simulink model "System_D_frequency_sweep"  (R2026a)
settings: Solver=ode23t  StopTime=1.45  MaxStep=1/(2*fs)  RelTol=1e-5
PostLoadFcn:
  | addpath(fileparts(get_param(bdroot,'FileName')));
InitFcn:
  | evalin('base','clear system_d_sweep_log system_d_frequency_response'); close(findall(groot,'Type','figure','Tag','SystemDFrequencyResponse'));
StopFcn:
  | plot_frequency_sweep(bdroot);
model workspace (MAT data in the model file):
  Cmid = 6.8e-06
  Ctw = 5.6e-06
  Lmid = 0.00082
  Ltw = 0.00022
  Rp = 3.3
  Rs = 4.7
  a_hp = [1 -1.96992019814 0.970365941122]
  a_lp = [1 -1.96992019814 0.970365941122]
  b_hp = [0.985071534816 -1.97014306963 0.985071534816]
  b_lp = [0.000111435745339 0.000222871490678 0.000111435745339]
  delay_samples = 16384
  f = [50 51 52 53 54 55 56 57 58 59 60 61 ... (412 elements, 412x1)]
  fir_mid = [2.88615785051e-06 2.87905807458e-06 2.86601289236e-06 2.86209989692e-06 2.87914488669e-06 2.90760278468e-06 2.91495292008e-06 2.86191467289e-06 2.72461541069e-06 2.51079055348e-06 2.26185413326e-06 2.03723101733e-06 ... (32768 elements, 1x32768)]
  fir_tw = [-2.60624232609e-06 -2.27215528381e-06 -2.25731305883e-06 -2.5961984087e-06 -2.98688820194e-06 -3.09958236215e-06 -2.8639414963e-06 -2.40425500843e-06 -1.83630123021e-06 -1.24253482671e-06 -7.49249289368e-07 -4.94473143896e-07 ... (32768 elements, 1x32768)]
  fir_woof = [2.71744577313e-06 2.91995199079e-06 3.2994659548e-06 3.73731262893e-06 4.11733049488e-06 4.36319861388e-06 4.44606576447e-06 4.38093146601e-06 4.22485207588e-06 4.06866670403e-06 4.00752757287e-06 4.09493136226e-06 ... (32768 elements, 1x32768)]
  fs = 96000
  g_woof = 0.595662143529
  pol_mid = 1
  pol_tw = 1
  pol_woof = 1
  ref_mid_im = [-2.02471473106e-05 -2.97451137892e-05 -8.18998441469e-06 -9.44112206059e-06 -9.98474521822e-06 -1.80323069699e-05 -2.36335585807e-05 -2.07669965717e-05 -2.44493768902e-05 1.53522925063e-05 1.26835054665e-05 -2.72017381443e-05 ... (412 elements, 412x1)]
  ref_mid_re = [5.11138743346e-05 5.27646175102e-05 6.43853406534e-05 7.19878043236e-05 9.07552490467e-05 9.02364974629e-05 0.000108111340774 0.000127641838401 0.000164076149146 0.00016525070791 0.000233272470596 0.000266015581949 ... (412 elements, 412x1)]
  ref_sum_im = [-0.237822623935 -0.249208923528 -0.252704050496 -0.277443609145 -0.287425433384 -0.281925307353 -0.273684166346 -0.301968651196 -0.32702532988 -0.356393021871 -0.384013551582 -0.427201303434 ... (412 elements, 412x1)]
  ref_sum_re = [0.0079461204201 -0.00807298700672 0.0366054479648 0.0304994442536 0.00185490294456 0.00396661293164 0.0289494720887 0.0412739478932 0.0471470600314 0.0668622907578 0.0743628077169 0.0739295887598 ... (412 elements, 412x1)]
  ref_tw_im = [2.66562025616e-10 1.06047214067e-10 3.29547259586e-10 9.1080418365e-11 1.01471933591e-10 -1.2721995912e-10 -3.07463357353e-10 -9.90286820009e-10 -4.40391607082e-10 -7.61622541983e-10 -4.0356932662e-10 2.86227803489e-10 ... (412 elements, 412x1)]
  ref_tw_re = [-2.81565378421e-10 4.5611348125e-11 -1.70188531961e-10 -5.4214307034e-11 1.59527809471e-12 1.81051243455e-11 4.85092069489e-10 1.65769684723e-11 -4.00879085044e-10 1.05530110859e-10 -9.04825296789e-10 -1.29396251722e-09 ... (412 elements, 412x1)]
  ref_woof_im = [-0.237802377054 -0.24917917852 -0.252695860841 -0.277434168114 -0.28741544874 -0.281907274919 -0.27366053248 -0.301947883209 -0.327000880063 -0.356408373402 -0.384026234684 -0.427174101982 ... (412 elements, 412x1)]
  ref_woof_re = [0.00789500682733 -0.00812575166984 0.0365410627943 0.0304274565035 0.00176414769392 0.00387637641607 0.0288413602628 0.0411463060382 0.0469829842831 0.0666970399443 0.0741295361511 0.0736635744718 ... (412 elements, 412x1)]
  sweep_input = [0 1.04166666667e-05 2.08333333333e-05 3.125e-05 4.16666666667e-05 5.20833333333e-05 6.25e-05 7.29166666667e-05 8.33333333333e-05 9.375e-05 0.000104166666667 0.000114583333333 ... (278402 elements, 139201x2)]
  tf_mid = [0.0998356483895 0.102076870231 0.0946421894936 0.0979510358274 0.112990905181 0.109044667147 0.122419200152 0.130377482303 0.15467322795 0.125179778541 0.168395608846 0.197284206678 ... (412 elements, 412x1)]
  tf_mid_im = [0.00966008754272 -0.00313844645705 0.0361663561834 0.0379690093634 0.0477044018154 0.03621348334 0.0393998382701 0.0511658321292 0.064682478583 0.0942375054511 0.119101574545 0.0996824269753 ... (412 elements, 412x1)]
  tf_mid_re = [0.0998356483895 0.102076870231 0.0946421894936 0.0979510358274 0.112990905181 0.109044667147 0.122419200152 0.130377482303 0.15467322795 0.125179778541 0.168395608846 0.197284206678 ... (412 elements, 412x1)]
  tf_tw = [0.0198457022563 8.34206280492e-05 0.012563148971 0.00336856881883 0.00145980497416 -0.00222599627599 -0.0157604599169 -0.0116189930625 0.00333344091506 -0.00916110563484 0.0108979357018 0.0209366637571 ... (412 elements, 412x1)]
  tf_tw_im = [-0.00715469241983 -0.00557696831399 -0.00982739097113 -0.00227734746733 -0.00315933910186 0.00326018180298 0.00155018479379 0.0216379610708 0.0128808016901 0.0125093739866 0.0144059793721 0.00636489608235 ... (412 elements, 412x1)]
  tf_tw_re = [0.0198457022563 8.34206280492e-05 0.012563148971 0.00336856881883 0.00145980497416 -0.00222599627599 -0.0157604599169 -0.0116189930625 0.00333344091506 -0.00916110563484 0.0108979357018 0.0209366637571 ... (412 elements, 412x1)]
  tf_woof = [0.181608417788 0.168786108916 0.242166050712 0.254795120302 0.223128594979 0.225804856879 0.259960687795 0.304360000511 0.337174588175 0.394426682217 0.432789825657 0.473682687703 ... (412 elements, 412x1)]
  tf_woof_im = [-0.356022917871 -0.383280529798 -0.354017107262 -0.393610885978 -0.428249167557 -0.416417838149 -0.382374342555 -0.411814390306 -0.441052500026 -0.464522244478 -0.494799805707 -0.553647303077 ... (412 elements, 412x1)]
  tf_woof_re = [0.181608417788 0.168786108916 0.242166050712 0.254795120302 0.223128594979 0.225804856879 0.259960687795 0.304360000511 0.337174588175 0.394426682217 0.432789825657 0.473682687703 ... (412 elements, 412x1)]
  zi_mid_im = [3.15145569017 3.226811686 3.32611598161 3.44333048105 3.54533776416 3.64854828115 3.76283446092 3.89289495957 4.01551140677 4.150592994 4.29260801654 4.46368784868 ... (412 elements, 412x1)]
  zi_mid_re = [5.31943483026 5.378404173 5.39638717148 5.47983267484 5.52299089563 5.59239183084 5.67547146448 5.74779130072 5.80510938691 5.884400566 5.98099909956 6.07160964327 ... (412 elements, 412x1)]
  zi_tw_im = [0.3929867032 0.3929867032 0.3929867032 0.3929867032 0.3929867032 0.3929867032 0.3929867032 0.3929867032 0.3929867032 0.3929867032 0.3929867032 0.3929867032 ... (412 elements, 412x1)]
  zi_tw_re = [3.639639303 3.639639303 3.639639303 3.639639303 3.639639303 3.639639303 3.639639303 3.639639303 3.639639303 3.639639303 3.639639303 3.639639303 ... (412 elements, 412x1)]
libraries: fl_lib x25, nesl_utility x5
(part 2 of 2)

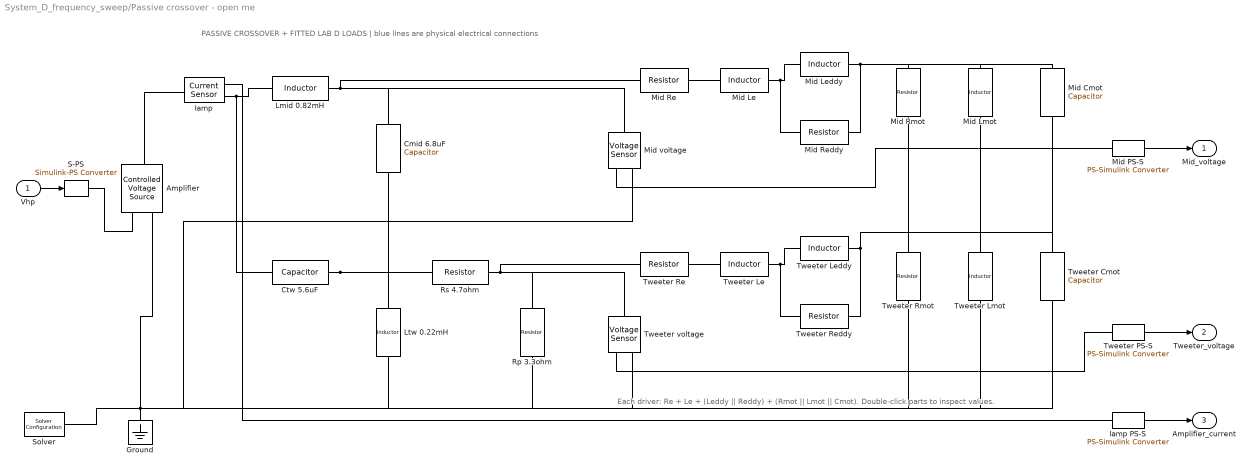
== system System_D_frequency_sweep/Passive crossover - open me ==
  note: PASSIVE CROSSOVER + FITTED LAB D LOADS | blue lines are physical electrical connections
  note: Each driver: Re + Le + (Leddy || Reddy) + (Rmot || Lmot || Cmot). Double-click parts to inspect values.
  Vhp : Inport
  Amplifier : fl_lib/Electrical/Electrical Sources/Controlled Voltage Source
  Cmid 6.8uF : fl_lib/Electrical/Electrical Elements/Capacitor  c=6.8e-06 F  r=0 Ohm  g=0 1/Ohm  i_specify=off  i_priority=None  i=0 A  i_nominal_specify=off  i_nominal_value=1  i_nominal_unit=A  v_specify=off  v_priority=None  v=0 V  v_nominal_specify=off  v_nominal_value=1  v_nominal_unit=V  vc_specify=off  vc_priority=High  vc=0 V  vc_nominal_specify=off  vc_nominal_value=1  vc_nominal_unit=V
  Ctw 5.6uF : fl_lib/Electrical/Electrical Elements/Capacitor  c=5.6e-06 F  r=0 Ohm  g=0 1/Ohm  i_specify=off  i_priority=None  i=0 A  i_nominal_specify=off  i_nominal_value=1  i_nominal_unit=A  v_specify=off  v_priority=None  v=0 V  v_nominal_specify=off  v_nominal_value=1  v_nominal_unit=V  vc_specify=off  vc_priority=High  vc=0 V  vc_nominal_specify=off  vc_nominal_value=1  vc_nominal_unit=V
  Ground : fl_lib/Electrical/Electrical Elements/Electrical Reference
  Iamp : fl_lib/Electrical/Electrical Sensors/Current Sensor
  Iamp PS-S : nesl_utility/PS-Simulink Converter  PhysicalDomain=network_engine_domain  SubClassName=ps_output  LeftPortType=input  RightPortType=output  PseudoPeriodic=off  Frequencies=[]  VectorFormat=inherit  Unit=A  AffineConversion=off
  Lmid 0.82mH : fl_lib/Electrical/Electrical Elements/Inductor  l=0.00082 H  r=0 Ohm  g=0 1/Ohm  i_specify=off  i_priority=None  i=0 A  i_nominal_specify=off  i_nominal_value=1  i_nominal_unit=A  v_specify=off  v_priority=None  v=0 V  v_nominal_specify=off  v_nominal_value=1  v_nominal_unit=V  i_L_specify=off  i_L_priority=High  i_L=0 A  i_L_nominal_specify=off  i_L_nominal_value=1  i_L_nominal_unit=A
  Ltw 0.22mH : fl_lib/Electrical/Electrical Elements/Inductor  l=0.00022 H  r=0 Ohm  g=0 1/Ohm  i_specify=off  i_priority=None  i=0 A  i_nominal_specify=off  i_nominal_value=1  i_nominal_unit=A  v_specify=off  v_priority=None  v=0 V  v_nominal_specify=off  v_nominal_value=1  v_nominal_unit=V  i_L_specify=off  i_L_priority=High  i_L=0 A  i_L_nominal_specify=off  i_L_nominal_value=1  i_L_nominal_unit=A
  Mid Cmot : fl_lib/Electrical/Electrical Elements/Capacitor  c=0.0004788 F  r=0 Ohm  g=0 1/Ohm  i_specify=off  i_priority=None  i=0 A  i_nominal_specify=off  i_nominal_value=1  i_nominal_unit=A  v_specify=off  v_priority=None  v=0 V  v_nominal_specify=off  v_nominal_value=1  v_nominal_unit=V  vc_specify=off  vc_priority=High  vc=0 V  vc_nominal_specify=off  vc_nominal_value=1  vc_nominal_unit=V
  Mid Le : fl_lib/Electrical/Electrical Elements/Inductor  l=0.0001699 H  r=0 Ohm  g=0 1/Ohm  i_specify=off  i_priority=None  i=0 A  i_nominal_specify=off  i_nominal_value=1  i_nominal_unit=A  v_specify=off  v_priority=None  v=0 V  v_nominal_specify=off  v_nominal_value=1  v_nominal_unit=V  i_L_specify=off  i_L_priority=High  i_L=0 A  i_L_nominal_specify=off  i_L_nominal_value=1  i_L_nominal_unit=A
  Mid Leddy : fl_lib/Electrical/Electrical Elements/Inductor  l=0.0004073 H  r=0 Ohm  g=0 1/Ohm  i_specify=off  i_priority=None  i=0 A  i_nominal_specify=off  i_nominal_value=1  i_nominal_unit=A  v_specify=off  v_priority=None  v=0 V  v_nominal_specify=off  v_nominal_value=1  v_nominal_unit=V  i_L_specify=off  i_L_priority=High  i_L=0 A  i_L_nominal_specify=off  i_L_nominal_value=1  i_L_nominal_unit=A
  Mid Lmot : fl_lib/Electrical/Electrical Elements/Inductor  l=0.006600000000000001 H  r=0 Ohm  g=0 1/Ohm  i_specify=off  i_priority=None  i=0 A  i_nominal_specify=off  i_nominal_value=1  i_nominal_unit=A  v_specify=off  v_priority=None  v=0 V  v_nominal_specify=off  v_nominal_value=1  v_nominal_unit=V  i_L_specify=off  i_L_priority=High  i_L=0 A  i_L_nominal_specify=off  i_L_nominal_value=1  i_L_nominal_unit=A
  Mid PS-S : nesl_utility/PS-Simulink Converter  PhysicalDomain=network_engine_domain  SubClassName=ps_output  LeftPortType=input  RightPortType=output  PseudoPeriodic=off  Frequencies=[]  VectorFormat=inherit  Unit=V  AffineConversion=off
  Mid Re : fl_lib/Electrical/Electrical Elements/Resistor  R=4.6 Ohm  i_specify=off  i_priority=None  i=0 A  i_nominal_specify=off  i_nominal_value=1  i_nominal_unit=A  v_specify=off  v_priority=None  v=0 V  v_nominal_specify=off  v_nominal_value=1  v_nominal_unit=V
  Mid Reddy : fl_lib/Electrical/Electrical Elements/Resistor  R=8.974 Ohm  i_specify=off  i_priority=None  i=0 A  i_nominal_specify=off  i_nominal_value=1  i_nominal_unit=A  v_specify=off  v_priority=None  v=0 V  v_nominal_specify=off  v_nominal_value=1  v_nominal_unit=V
  Mid Rmot : fl_lib/Electrical/Electrical Elements/Resistor  R=14.21262080727686 Ohm  i_specify=off  i_priority=None  i=0 A  i_nominal_specify=off  i_nominal_value=1  i_nominal_unit=A  v_specify=off  v_priority=None  v=0 V  v_nominal_specify=off  v_nominal_value=1  v_nominal_unit=V
  Mid voltage : fl_lib/Electrical/Electrical Sensors/Voltage Sensor
  Rp 3.3ohm : fl_lib/Electrical/Electrical Elements/Resistor  R=3.3 Ohm  i_specify=off  i_priority=None  i=0 A  i_nominal_specify=off  i_nominal_value=1  i_nominal_unit=A  v_specify=off  v_priority=None  v=0 V  v_nominal_specify=off  v_nominal_value=1  v_nominal_unit=V
  Rs 4.7ohm : fl_lib/Electrical/Electrical Elements/Resistor  R=4.7 Ohm  i_specify=off  i_priority=None  i=0 A  i_nominal_specify=off  i_nominal_value=1  i_nominal_unit=A  v_specify=off  v_priority=None  v=0 V  v_nominal_specify=off  v_nominal_value=1  v_nominal_unit=V
  S-PS : nesl_utility/Simulink-PS Converter  PhysicalDomain=network_engine_domain  SubClassName=ps_input  LeftPortType=input  RightPortType=output  PseudoPeriodic=off  Frequencies=[]  NoiseDistribution=none  NoiseParameters=[]  Unit=V  AffineConversion=off  FilteringAndDerivatives=provide  SimscapeFilterOrder=1  InputFilterTimeConstant=0.001  UdotUserProvided=0
  Solver : nesl_utility/Solver Configuration  PhysicalDomain=network_engine_domain  SubClassName=solver  LeftPortType=input  RightPortType=generic  Tones=[]  Harmonics=[]  SimulateNoise=off  Profile=off  UseLocalSampling=off  EnableSwitchedLinearOptims=on  FrequencyDomain=off  UseCCode=off  RelTol=0.001  AbsTol=0.001  MinStep=1e-09  ToWorkspace=off  RevertToSquareIcSolve=off  NumHomotopyIterations=100  PhasorMode=off  PhasorModeNumHarmonics=1  ConsistencySolver=NEWTON_XTOL_AFTER_FTOL  CanonicalOrdering=CANONICAL  OptimizeIntermediates=OPTIMIZED  IndexReductionMethod=DerivativeReplacement  DoDC=off  ResidualTolerance=1e-09  ConsistencyTolSource=GLOBAL  ConsistencyAbsTol=0.001  ConsistencyRelTol=0.001  ConsistencyTolFactor=0.001  UseLocalSolver=off  LocalSolverChoice=NE_BACKWARD_EULER_ADVANCER  ResolveIndetEquations=on  FunctionEvalNumThread=1  LocalSolverSampleTime=0.001  DoFixedCost=off  MaxNonlinIter=3  MaxModeIter=2  ComputeImpulses=off  ImpulseIterations=2  LinearAlgebra=auto  LinearAlgebraNumThread=0  EquationFormulation=NE_TIME_EF  DelaysMemoryBudget=1024  AutomaticFiltering=on  FilteringTimeConstant=0.001  PartitionStorageMethod=AS_NEEDED  PartitionMemoryBudget=1024  PartitionMethod=ROBUST  MultibodyUseLocalSolver=off  MultibodyLocalSolverChoice=ODE1  MultibodyLocalSolverSampleTime=0.001
  Tweeter Cmot : fl_lib/Electrical/Electrical Elements/Capacitor  c=5.582222222222222e-05 F  r=0 Ohm  g=0 1/Ohm  i_specify=off  i_priority=None  i=0 A  i_nominal_specify=off  i_nominal_value=1  i_nominal_unit=A  v_specify=off  v_priority=None  v=0 V  v_nominal_specify=off  v_nominal_value=1  v_nominal_unit=V  vc_specify=off  vc_priority=High  vc=0 V  vc_nominal_specify=off  vc_nominal_value=1  vc_nominal_unit=V
  Tweeter Le : fl_lib/Electrical/Electrical Elements/Inductor  l=1.942e-05 H  r=0 Ohm  g=0 1/Ohm  i_specify=off  i_priority=None  i=0 A  i_nominal_specify=off  i_nominal_value=1  i_nominal_unit=A  v_specify=off  v_priority=None  v=0 V  v_nominal_specify=off  v_nominal_value=1  v_nominal_unit=V  i_L_specify=off  i_L_priority=High  i_L=0 A  i_L_nominal_specify=off  i_L_nominal_value=1  i_L_nominal_unit=A
  Tweeter Leddy : fl_lib/Electrical/Electrical Elements/Inductor  l=2.364e-05 H  r=0 Ohm  g=0 1/Ohm  i_specify=off  i_priority=None  i=0 A  i_nominal_specify=off  i_nominal_value=1  i_nominal_unit=A  v_specify=off  v_priority=None  v=0 V  v_nominal_specify=off  v_nominal_value=1  v_nominal_unit=V  i_L_specify=off  i_L_priority=High  i_L=0 A  i_L_nominal_specify=off  i_L_nominal_value=1  i_L_nominal_unit=A
  Tweeter Lmot : fl_lib/Electrical/Electrical Elements/Inductor  l=0.00022455 H  r=0 Ohm  g=0 1/Ohm  i_specify=off  i_priority=None  i=0 A  i_nominal_specify=off  i_nominal_value=1  i_nominal_unit=A  v_specify=off  v_priority=None  v=0 V  v_nominal_specify=off  v_nominal_value=1  v_nominal_unit=V  i_L_specify=off  i_L_priority=High  i_L=0 A  i_L_nominal_specify=off  i_L_nominal_value=1  i_L_nominal_unit=A
  Tweeter PS-S : nesl_utility/PS-Simulink Converter  PhysicalDomain=network_engine_domain  SubClassName=ps_output  LeftPortType=input  RightPortType=output  PseudoPeriodic=off  Frequencies=[]  VectorFormat=inherit  Unit=V  AffineConversion=off
  Tweeter Re : fl_lib/Electrical/Electrical Elements/Resistor  R=3.4 Ohm  i_specify=off  i_priority=None  i=0 A  i_nominal_specify=off  i_nominal_value=1  i_nominal_unit=A  v_specify=off  v_priority=None  v=0 V  v_nominal_specify=off  v_nominal_value=1  v_nominal_unit=V
  Tweeter Reddy : fl_lib/Electrical/Electrical Elements/Resistor  R=1.577 Ohm  i_specify=off  i_priority=None  i=0 A  i_nominal_specify=off  i_nominal_value=1  i_nominal_unit=A  v_specify=off  v_priority=None  v=0 V  v_nominal_specify=off  v_nominal_value=1  v_nominal_unit=V
  Tweeter Rmot : fl_lib/Electrical/Electrical Elements/Resistor  R=3.106662064204349 Ohm  i_specify=off  i_priority=None  i=0 A  i_nominal_specify=off  i_nominal_value=1  i_nominal_unit=A  v_specify=off  v_priority=None  v=0 V  v_nominal_specify=off  v_nominal_value=1  v_nominal_unit=V
  Tweeter voltage : fl_lib/Electrical/Electrical Sensors/Voltage Sensor
  Mid_voltage : Outport
  Tweeter_voltage : Outport  Port=2
  Amplifier_current : Outport  Port=3
  wires:
  Vhp/1 -> S-PS/1
  Mid PS-S/1 -> Mid_voltage/1
  Tweeter PS-S/1 -> Tweeter_voltage/1
  Iamp PS-S/1 -> Amplifier_current/1
  connections:
  Amplifier/RConn2 -- Tweeter voltage/RConn2 -- Ground/LConn1 -- Tweeter Cmot/RConn1 -- Tweeter Lmot/RConn1 -- Tweeter Rmot/RConn1 -- Mid voltage/RConn2 -- Mid Cmot/RConn1 -- Mid Lmot/RConn1 -- Mid Rmot/RConn1 -- Rp 3.3ohm/RConn1 -- Ltw 0.22mH/RConn1 -- Cmid 6.8uF/RConn1 -- Solver/RConn1
  Iamp/RConn2 -- Ctw 5.6uF/LConn1 -- Lmid 0.82mH/LConn1
  Lmid 0.82mH/RConn1 -- Mid voltage/LConn1 -- Mid Re/LConn1 -- Cmid 6.8uF/LConn1
  Ctw 5.6uF/RConn1 -- Rs 4.7ohm/LConn1 -- Ltw 0.22mH/LConn1
  Rs 4.7ohm/RConn1 -- Tweeter voltage/LConn1 -- Tweeter Re/LConn1 -- Rp 3.3ohm/LConn1
  Mid Le/RConn1 -- Mid Reddy/LConn1 -- Mid Leddy/LConn1
  Mid Leddy/RConn1 -- Mid Cmot/LConn1 -- Mid Lmot/LConn1 -- Mid Rmot/LConn1 -- Mid Reddy/RConn1
  Tweeter Le/RConn1 -- Tweeter Reddy/LConn1 -- Tweeter Leddy/LConn1
  Tweeter Leddy/RConn1 -- Tweeter Cmot/LConn1 -- Tweeter Lmot/LConn1 -- Tweeter Rmot/LConn1 -- Tweeter Reddy/RConn1
  S-PS/RConn1 -- Amplifier/RConn1
  Amplifier/LConn1 -- Iamp/LConn1
  Mid Re/RConn1 -- Mid Le/LConn1
  Mid voltage/RConn1 -- Mid PS-S/LConn1
  Tweeter Re/RConn1 -- Tweeter Le/LConn1
  Tweeter voltage/RConn1 -- Tweeter PS-S/LConn1
  Iamp/RConn1 -- Iamp PS-S/LConn1
